simulink model "kalman_cv"  (R2025b)
settings: Solver=FixedStepDiscrete  StartTime=0.0  StopTime=20  FixedStep=0.1  RelTol=1e-3
settings Model: Creator=alosw  LastModifiedBy=alosw

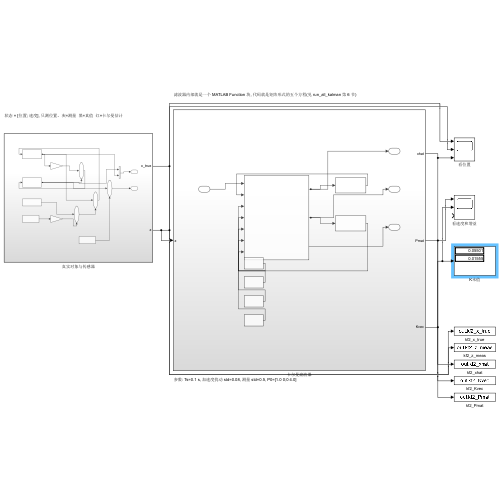
[thumbnail: Simulink's stored preview of the top-level diagram]
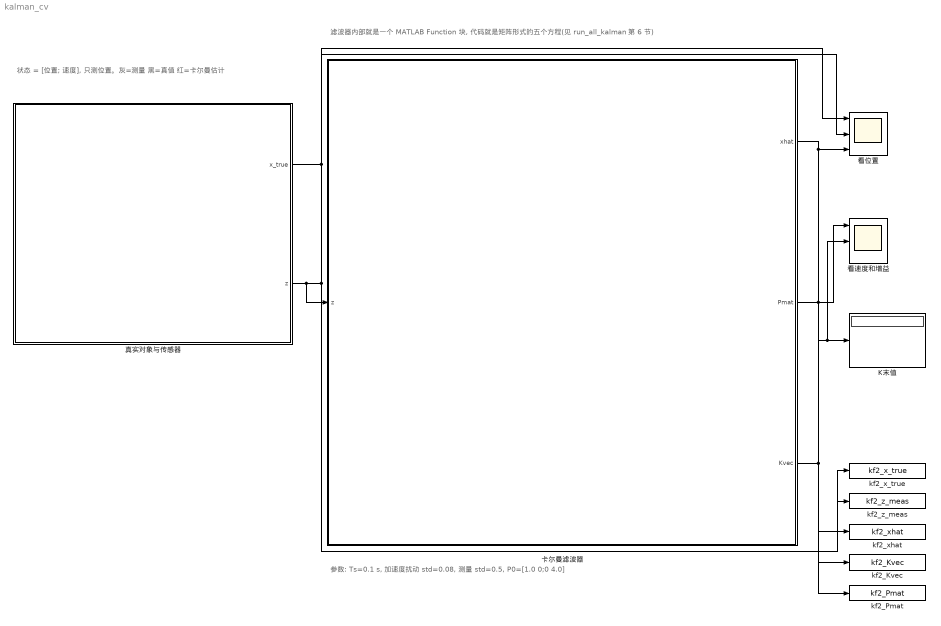
== system kalman_cv ==
  note: 状态 = [位置; 速度], 只测位置。灰=测量 黑=真值 红=卡尔曼估计
  note: 滤波器内部就是一个 MATLAB Function 块, 代码就是矩阵形式的五个方程(见 run_all_kalman 第 6 节)
  note: 参数: Ts=0.1 s, 加速度扰动 std=0.08, 测量 std=0.5, P0=[1.0 0;0 4.0]
  K末值 : Display
  kf2_Kvec : ToWorkspace  VariableName=kf2_Kvec  SaveFormat=Timeseries  SampleTime=-1
  kf2_Pmat : ToWorkspace  VariableName=kf2_Pmat  SaveFormat=Timeseries  SampleTime=-1
  kf2_x_true : ToWorkspace  VariableName=kf2_x_true  SaveFormat=Timeseries  SampleTime=-1
  kf2_xhat : ToWorkspace  VariableName=kf2_xhat  SaveFormat=Timeseries  SampleTime=-1
  kf2_z_meas : ToWorkspace  VariableName=kf2_z_meas  SaveFormat=Timeseries  SampleTime=-1
  卡尔曼滤波器 : Subsystem
  看位置 : Scope  NumInputPorts=3
      settings: ActiveDisplayYMinimum=-12.344087182842411  ActiveDisplayYMaximum=6.4551951164094712
  看速度和增益 : Scope  NumInputPorts=3
      settings: ActiveDisplayYMinimum=-0.12929442743123404  ActiveDisplayYMaximum=1.3014596855008498
  真实对象与传感器 : Subsystem
  wires:
  真实对象与传感器/1(x_true) -> 看位置/1, kf2_x_true/1
  真实对象与传感器/2(z) -> 看位置/2, kf2_z_meas/1, 卡尔曼滤波器/1(z)
  卡尔曼滤波器/1(xhat) -> kf2_xhat/1, 看位置/3
  卡尔曼滤波器/2(Pmat) -> 看速度和增益/1, kf2_Pmat/1
  卡尔曼滤波器/3(Kvec) -> K末值/1, 看速度和增益/2, kf2_Kvec/1

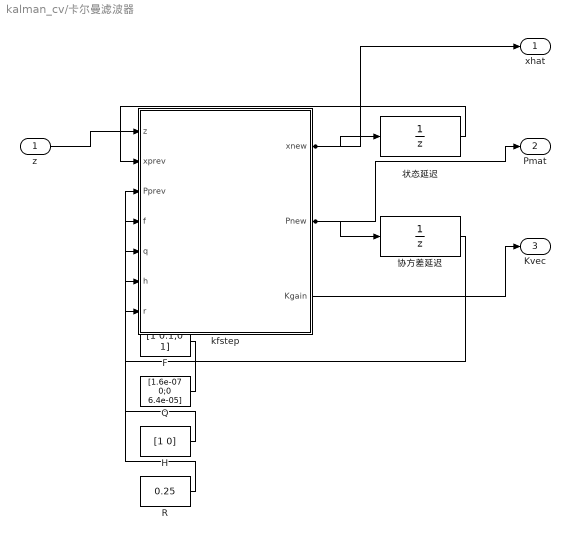
== system kalman_cv/卡尔曼滤波器 ==
  z : Inport
  F : Constant  Value=[1 0.1;0 1]  OutDataTypeStr=double
  H : Constant  Value=[1 0]  OutDataTypeStr=double
  Q : Constant  Value=[1.6e-07 0;0 6.4e-05]  OutDataTypeStr=double
  R : Constant  Value=0.25  OutDataTypeStr=double
  kfstep : MATLAB Function  TreatAsAtomicUnit=on
  协方差延迟 : UnitDelay  InitialCondition=[1 0;0 4]  SampleTime=0.1  HasFrameUpgradeWarning=on
  状态延迟 : UnitDelay  InitialCondition=[0;0]  SampleTime=0.1  HasFrameUpgradeWarning=on
  xhat : Outport
  Pmat : Outport  Port=2
  Kvec : Outport  Port=3
  wires:
  z/1 -> kfstep/1(z)
  状态延迟/1 -> kfstep/2(xprev)
  协方差延迟/1 -> kfstep/3(Pprev)
  F/1 -> kfstep/4(f)
  Q/1 -> kfstep/5(q)
  H/1 -> kfstep/6(h)
  R/1 -> kfstep/7(r)
  kfstep/1(xnew) -> 状态延迟/1, xhat/1
  kfstep/2(Pnew) -> 协方差延迟/1, Pmat/1
  kfstep/3(Kgain) -> Kvec/1

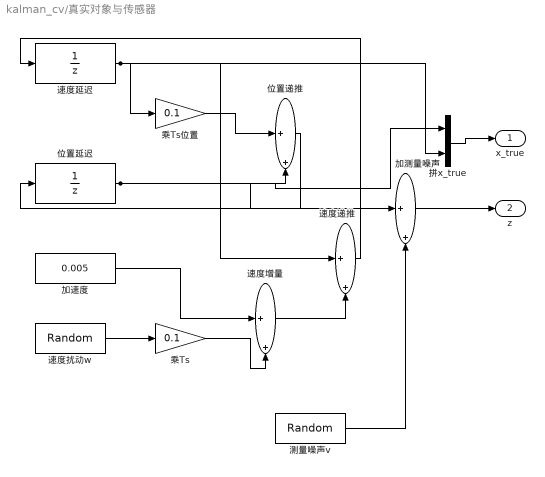
== system kalman_cv/真实对象与传感器 ==
  乘Ts : Gain  Gain=0.1
  乘Ts位置 : Gain  Gain=0.1
  位置延迟 : UnitDelay  SampleTime=0.1  HasFrameUpgradeWarning=on
  位置递推 : Sum  Inputs=|++
  加测量噪声 : Sum  Inputs=|++
  加速度 : Constant  Value=0.005  OutDataTypeStr=double
  拼x_true : Mux  Inputs=2
  测量噪声v : RandomNumber  Variance=0.25  Seed=777  SampleTime=0.1
  速度增量 : Sum  Inputs=|++
  速度延迟 : UnitDelay  InitialCondition=-1.4  SampleTime=0.1  HasFrameUpgradeWarning=on
  速度扰动w : RandomNumber  Variance=0.0064  Seed=2026  SampleTime=0.1
  速度递推 : Sum  Inputs=|++
  x_true : Outport
  z : Outport  Port=2
  wires:
  速度延迟/1 -> 乘Ts位置/1, 速度递推/1, 拼x_true/2
  乘Ts位置/1 -> 位置递推/1
  位置延迟/1 -> 位置递推/2, 加测量噪声/1, 拼x_true/1
  位置递推/1 -> 位置延迟/1
  加速度/1 -> 速度增量/1
  速度扰动w/1 -> 乘Ts/1
  乘Ts/1 -> 速度增量/2
  速度增量/1 -> 速度递推/2
  速度递推/1 -> 速度延迟/1
  测量噪声v/1 -> 加测量噪声/2
  拼x_true/1 -> x_true/1
  加测量噪声/1 -> z/1

== matlab function kalman_cv/卡尔曼滤波器/kfstep ==
  data: z input double size=[1 1]; xprev input double size=[2 1]; Pprev input double size=[2 2]; f input double size=[2 2]; q input double size=[2 2]; h input double size=[1 2]; r input double size=[1 1]; xnew output double size=[2 1]; Pnew output double size=[2 2]; Kgain output double size=[2 1]
function [xnew, Pnew, Kgain] = fcn(z, xprev, Pprev, f, q, h, r)
xp = f*xprev;
Pp = f*Pprev*f' + q;
S  = h*Pp*h' + r;
Kgain = Pp*h'/S;
xnew = xp + Kgain*(z - h*xp);
Pnew = (eye(2) - Kgain*h)*Pp;
